simulink model "KneeTransient"  (R2025a)
settings: Solver=ode45  StartTime=0.0  StopTime=50  MaxStep=0.001  RelTol=1e-8  AbsTol=1e-10
PreLoadFcn:
  | I_knee = 0.06;      % kg*m^2 below-knee inertia (rig estimate)
  | b_knee = 0.5;        % N*m*s/rad joint damping
  | K_knee = 0.5;       % N*m/rad return spring
  | th0    = 0.26;      % rad spring rest angle (~15 deg)
  | ROM    = 1.5708;    % rad (90 deg) normalizing range
  | r_arm  = 0.035;     % m BPA moment arm
  | Tload  = 0.5;       % N*m constant flexion load torque
  | desc_ext = 4.2;     % nA descending drive to extensor MN
  | desc_flex = 2.5;    % nA descending drive to flexor MN
  | Fmax_ext = 500;     % N
  | Fmax_flex = 450;    % N
  | epsScale = 0.15;    % muscle strain span over full joint ROM
  | tapAmplitude=2;
libraries: SNS_Library x20
settings Model: Creator=Ben Bolen  LastModifiedBy=Ben Bolen

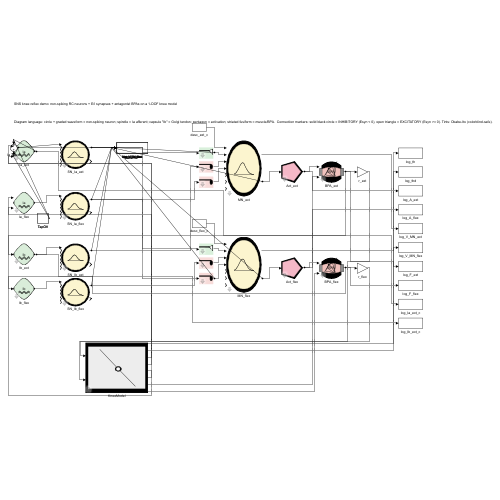
[thumbnail: Simulink's stored preview of the top-level diagram]
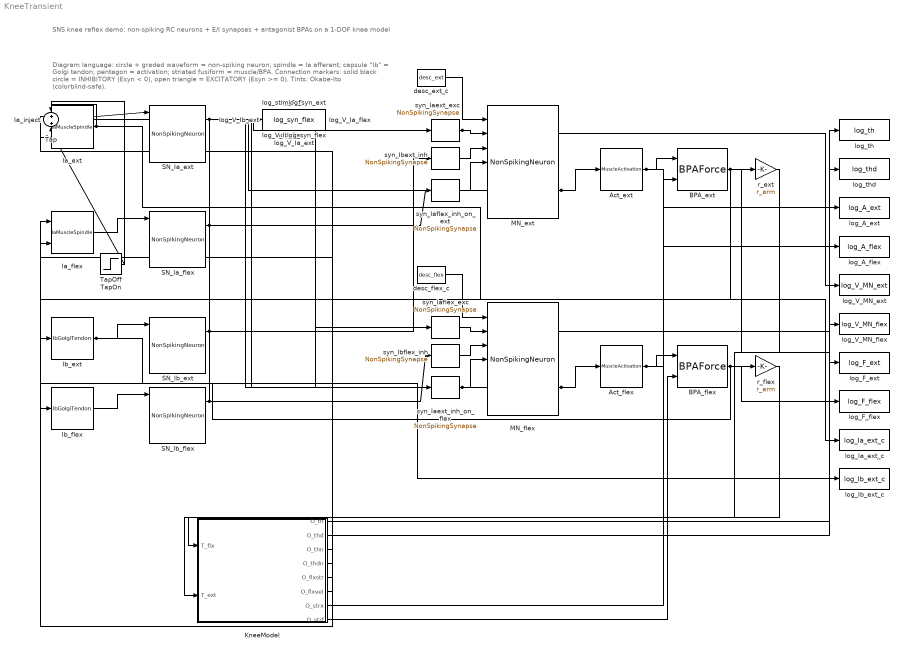
== system KneeTransient ==
  note: SNS knee reflex demo: non-spiking RC neurons + E/I synapses + antagonist BPAs on a 1-DOF knee model
  note: Diagram language: circle + graded waveform = non-spiking neuron; spindle = Ia afferent; capsule "Ib" = Golgi tendon; pentagon = activation; striated fusiform = muscle/BPA. Connection markers: solid black circle = INHIBITORY (Esyn < 0), open triangle = EXCITATORY (Esyn >= 0). Tints: Okabe-Ito (colorblind-safe).
  Act_ext : SNS_Library/MuscleActivation  tauAct=50  A0=0
  Act_flex : SNS_Library/MuscleActivation  tauAct=50  A0=0
  BPA_ext : SNS_Library/BPAForce  Fmax=Fmax_ext  epsMax=0.25
  BPA_flex : SNS_Library/BPAForce  Fmax=Fmax_flex  epsMax=0.25
  Ia_ext : SNS_Library/IaMuscleSpindle  Imax=10  Wl=6  Wv=8
  Ia_flex : SNS_Library/IaMuscleSpindle  Imax=10  Wl=6  Wv=8
  Ia_inject : Sum
  Ib_ext : SNS_Library/IbGolgiTendon  Imax=10  Kf=0.02
  Ib_flex : SNS_Library/IbGolgiTendon  Imax=10  Kf=0.0222
  KneeModel : Subsystem  mask(SNS Knee Model (1-DOF)){}
      mask help: Reduced-order 1-DOF knee: I*thdd = Tflex - Text + Tload - b*thd - K*(th-th0). theta = 0 deg full extension, +90 deg full flexion. Outputs theta, thd, and the normalized stretch/velocity/strain signals for the afferents.
      mask Display:
      | patch([-1 1 1 -1], [-1 -1 1 1], [0 0 0]);
      | patch([-0.92 0.92 0.92 -0.92], [-0.84 -0.84 0.84 0.84], [0.93 0.93 0.93]);
      | color('black');
      | plot([-0.55 0.05], [0.75 -0.05]);
      | plot([0.05 0.60], [-0.05 -0.75]);
      | t_ = linspace(0, 2*pi, 25);
      | patch(0.10*cos(t_) + 0.05, 0.10*sin(t_) - 0.05, [0 0 0]);
      | patch(0.055*cos(t_) + 0.05, 0.055*sin(t_) - 0.05, [1 1 1]);
  MN_ext : SNS_Library/NonSpikingNeuron  Vrest=-52  Gm=0.5  Cm=2.5  Thr=-45  Slope=10
  MN_flex : SNS_Library/NonSpikingNeuron  Vrest=-52  Gm=0.5  Cm=2.5  Thr=-45  Slope=10
  SN_Ia_ext : SNS_Library/NonSpikingNeuron  Vrest=-52  Gm=0.4  Cm=2  Thr=-55  Slope=1
  SN_Ia_flex : SNS_Library/NonSpikingNeuron  Vrest=-52  Gm=0.4  Cm=2  Thr=-55  Slope=1
  SN_Ib_ext : SNS_Library/NonSpikingNeuron  Vrest=-52  Gm=0.4  Cm=2  Thr=-55  Slope=1
  SN_Ib_flex : SNS_Library/NonSpikingNeuron  Vrest=-52  Gm=0.4  Cm=2  Thr=-55  Slope=1
  Tap : Sum
  TapOff : Step  Time=30.03  After=-tapAmplitude  SampleTime=0
  TapOn : Step  Time=30  After=tapAmplitude  SampleTime=0
  desc_ext_c : Constant  Value=desc_ext
  desc_flex_c : Constant  Value=desc_flex
  log_A_ext : ToWorkspace  VariableName=log_A_ext  SaveFormat=Timeseries  SampleTime=-1
  log_A_flex : ToWorkspace  VariableName=log_A_flex  SaveFormat=Timeseries  SampleTime=-1
  log_F_ext : ToWorkspace  VariableName=log_F_ext  SaveFormat=Timeseries  SampleTime=-1
  log_F_flex : ToWorkspace  VariableName=log_F_flex  SaveFormat=Timeseries  SampleTime=-1
  log_Ia_ext_c : ToWorkspace  VariableName=log_Ia_ext_c  SaveFormat=Timeseries  SampleTime=-1
  log_Ib_ext_c : ToWorkspace  VariableName=log_Ib_ext_c  SaveFormat=Timeseries  SampleTime=-1
  log_S_ext : ToWorkspace  VariableName=log_S_ext  SaveFormat=Timeseries  SampleTime=-1
  log_S_flex : ToWorkspace  VariableName=log_S_flex  SaveFormat=Timeseries  SampleTime=-1
  log_V_Ia_ext : ToWorkspace  VariableName=log_V_Ia_ext  SaveFormat=Timeseries  SampleTime=-1
  log_V_Ia_flex : ToWorkspace  VariableName=log_V_Ia_flex  SaveFormat=Timeseries  SampleTime=-1
  log_V_Ib_ext : ToWorkspace  VariableName=log_V_Ib_ext  SaveFormat=Timeseries  SampleTime=-1
  log_V_Ib_flex : ToWorkspace  VariableName=log_V_Ib_flex  SaveFormat=Timeseries  SampleTime=-1
  log_V_MN_ext : ToWorkspace  VariableName=log_V_MN_ext  SaveFormat=Timeseries  SampleTime=-1
  log_V_MN_flex : ToWorkspace  VariableName=log_V_MN_flex  SaveFormat=Timeseries  SampleTime=-1
  log_stim : ToWorkspace  VariableName=log_stim  SaveFormat=Timeseries  SampleTime=-1
  log_syn_ext : ToWorkspace  VariableName=log_syn_ext  SaveFormat=Timeseries  SampleTime=-1
  log_syn_flex : ToWorkspace  VariableName=log_syn_flex  SaveFormat=Timeseries  SampleTime=-1
  log_th : ToWorkspace  VariableName=log_th  SaveFormat=Timeseries  SampleTime=-1
  log_thd : ToWorkspace  VariableName=log_thd  SaveFormat=Timeseries  SampleTime=-1
  r_ext : Gain  Gain=r_arm
  r_flex : Gain  Gain=r_arm
  syn_Iaext_exc : SNS_Library/NonSpikingSynapse  gmax=0.18  Esyn=0  ThrPre=-45  SlopePre=10
  syn_Iaext_inh_on_flex : SNS_Library/NonSpikingSynapse  gmax=0.15  Esyn=-72  ThrPre=-45  SlopePre=10
  syn_Iaflex_exc : SNS_Library/NonSpikingSynapse  gmax=0.18  Esyn=0  ThrPre=-45  SlopePre=10
  syn_Iaflex_inh_on_ext : SNS_Library/NonSpikingSynapse  gmax=0.15  Esyn=-72  ThrPre=-45  SlopePre=10
  syn_Ibext_inh : SNS_Library/NonSpikingSynapse  gmax=0.20  Esyn=-72  ThrPre=-45  SlopePre=0.5
  syn_Ibflex_inh : SNS_Library/NonSpikingSynapse  gmax=0.20  Esyn=-72  ThrPre=-45  SlopePre=0.5
  wires:
  KneeModel/3(O_thn) -> Ia_ext/1
  KneeModel/4(O_thdn) -> Ia_ext/2
  KneeModel/5(O_flxstr) -> Ia_flex/1
  KneeModel/6(O_flxvel) -> Ia_flex/2
  Ia_ext/1 -> log_Ia_ext_c/1, Ia_inject/1
  Ia_flex/1 -> SN_Ia_flex/1
  Ib_ext/1 -> SN_Ib_ext/1, log_Ib_ext_c/1
  Ib_flex/1 -> SN_Ib_flex/1
  desc_ext_c/1 -> MN_ext/1
  desc_flex_c/1 -> MN_flex/1
  SN_Ia_ext/1 -> syn_Iaext_exc/1, syn_Iaext_inh_on_flex/1, log_V_Ia_ext/1
  SN_Ib_ext/1 -> syn_Ibext_inh/1, log_V_Ib_ext/1
  SN_Ia_flex/1 -> syn_Iaflex_inh_on_ext/1, syn_Iaflex_exc/1, log_V_Ia_flex/1
  SN_Ib_flex/1 -> syn_Ibflex_inh/1, log_V_Ib_flex/1
  syn_Iaext_exc/1 -> MN_ext/2, log_syn_ext/1
  syn_Ibext_inh/1 -> MN_ext/3
  syn_Iaflex_inh_on_ext/1 -> MN_ext/4
  syn_Iaflex_exc/1 -> MN_flex/2
  syn_Ibflex_inh/1 -> MN_flex/3
  syn_Iaext_inh_on_flex/1 -> MN_flex/4, log_syn_flex/1
  MN_ext/2 -> Act_ext/1, log_S_ext/1
  MN_flex/2 -> Act_flex/1, log_S_flex/1
  Act_ext/1 -> BPA_ext/1, log_A_ext/1
  Act_flex/1 -> BPA_flex/1, log_A_flex/1
  KneeModel/7(O_strx) -> BPA_ext/2
  KneeModel/8(O_strf) -> BPA_flex/2
  BPA_ext/1 -> Ib_ext/1, r_ext/1, log_F_ext/1
  BPA_flex/1 -> Ib_flex/1, r_flex/1, log_F_flex/1
  r_flex/1 -> KneeModel/1(T_flx)
  r_ext/1 -> KneeModel/2(T_ext)
  KneeModel/1(O_th) -> log_th/1
  KneeModel/2(O_thd) -> log_thd/1
  MN_ext/1 -> log_V_MN_ext/1
  MN_flex/1 -> log_V_MN_flex/1
  TapOn/1 -> Tap/1
  TapOff/1 -> Tap/2
  Tap/1 -> Ia_inject/2, log_stim/1
  Ia_inject/1 -> SN_Ia_ext/1

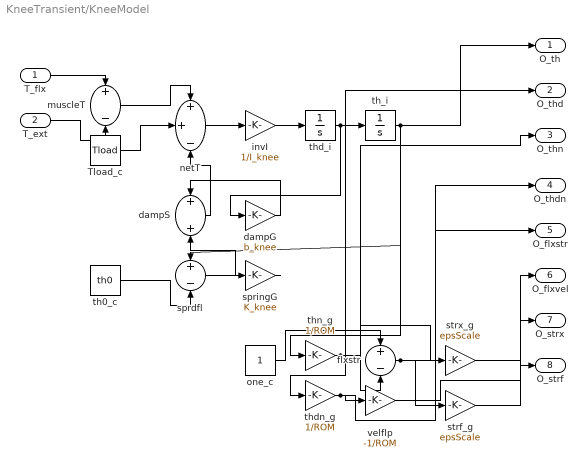
== system KneeTransient/KneeModel ==
  T_flx : Inport
  T_ext : Inport  Port=2
  Tload_c : Constant  Value=Tload
  dampG : Gain  Gain=b_knee
  dampS : Sum
  flxstr : Sum  Inputs=+-
  invI : Gain  Gain=1/I_knee
  muscleT : Sum  Inputs=+-
  netT : Sum  Inputs=++-
  one_c : Constant
  sprdfl : Sum  Inputs=+-
  springG : Gain  Gain=K_knee
  strf_g : Gain  Gain=epsScale
  strx_g : Gain  Gain=epsScale
  th0_c : Constant  Value=th0
  th_i : Integrator  InitialCondition=0.26
  thd_i : Integrator
  thdn_g : Gain  Gain=1/ROM
  thn_g : Gain  Gain=1/ROM
  velflp : Gain  Gain=-1/ROM
  O_th : Outport
  O_thd : Outport  Port=2
  O_thn : Outport  Port=3
  O_thdn : Outport  Port=4
  O_flxstr : Outport  Port=5
  O_flxvel : Outport  Port=6
  O_strx : Outport  Port=7
  O_strf : Outport  Port=8
  wires:
  T_flx/1 -> muscleT/1
  T_ext/1 -> muscleT/2
  muscleT/1 -> netT/1
  Tload_c/1 -> netT/2
  dampS/1 -> netT/3
  netT/1 -> invI/1
  invI/1 -> thd_i/1
  thd_i/1 -> th_i/1, dampG/1, O_thd/1, thdn_g/1
  th_i/1 -> sprdfl/1, O_th/1, thn_g/1
  th0_c/1 -> sprdfl/2
  sprdfl/1 -> springG/1
  dampG/1 -> dampS/1
  springG/1 -> dampS/2
  thn_g/1 -> O_thn/1, flxstr/2, strx_g/1
  thdn_g/1 -> O_thdn/1, velflp/1
  one_c/1 -> flxstr/1
  flxstr/1 -> O_flxstr/1, strf_g/1
  velflp/1 -> O_flxvel/1
  strx_g/1 -> O_strx/1
  strf_g/1 -> O_strf/1
